simulink model "Es_stateflow"  (R2025b)
settings: Solver=VariableStepAuto  StartTime=0.0  StopTime=10.0  RelTol=1e-3
settings Model: Creator=fsisa  LastModifiedBy=fsisa

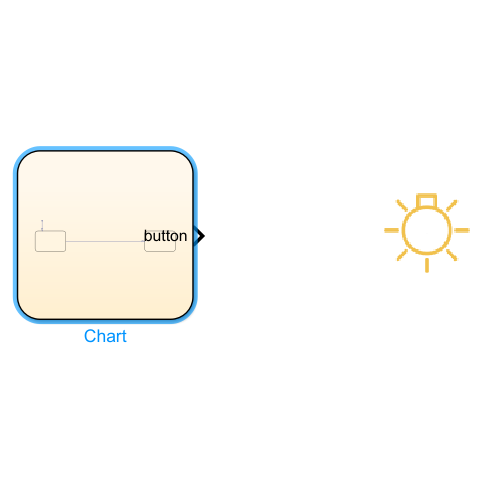
[thumbnail: Simulink's stored preview of the top-level diagram]
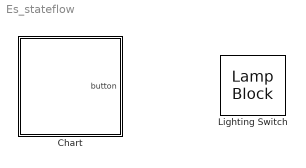
== system Es_stateflow ==
  Chart : Stateflow chart  TreatAsAtomicUnit=on
  Lighting Switch : LampBlock  LabelPosition=Hide  DefaultColor=[192.0, 192.0, 192.0]  Icon=LightingSwitch

== stateflow chart Es_stateflow/Chart ==
  state OFF
    entry:
    button=0;
  state ON
    entry:
    button=1;
  (default) -> OFF
  OFF -> ON : after(5,sec)
  data: button output; data local
